simulink library "casper_library_delays"  (Simulink 7.2)
settings: Solver=ode45  SolverMode=SingleTasking  StartTime=0.0  StopTime=10.0  RelTol=1e-3
libraries: xbsIndex_r4 x388, casper_library_misc x16, casper_library_delays x16, xbsReplacements_r4 x5, casper_library_multipliers x4
(part 2 of 5)

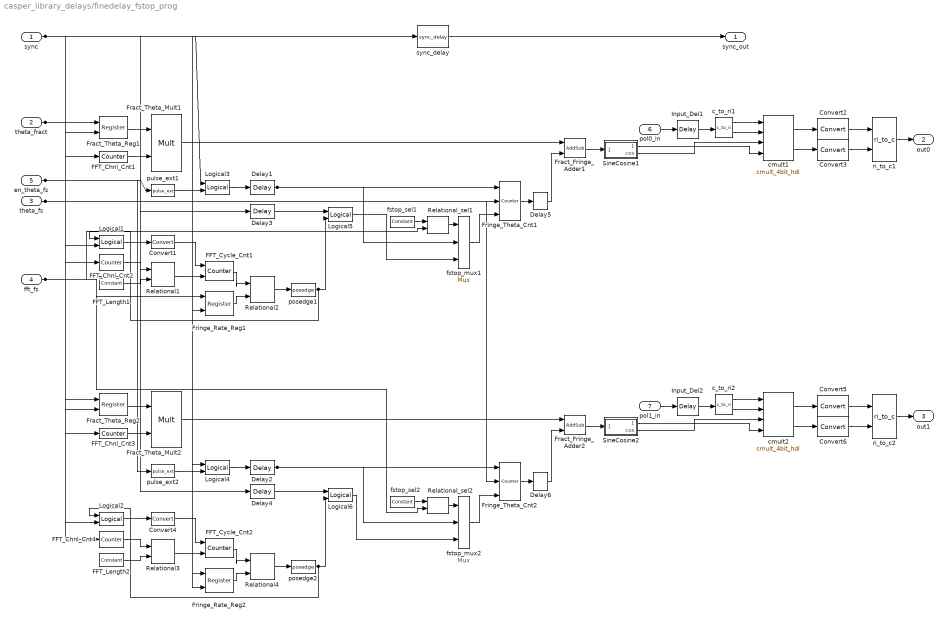
== system casper_library_delays/finedelay_fstop_prog ==
  sync : Inport
  theta_fract : Inport  Port=2
  theta_fs : Inport  Port=3
  fft_fs : Inport  Port=4
  en_theta_fs : Inport  Port=5
  pol0_in : Inport  Port=6
  pol1_in : Inport  Port=7
  Convert1 : xbsIndex_r4/Convert  gui_display_data_type=Fixed-point  arith_type=Boolean  n_bits=16  bin_pt=14  float_type=Single  exp_bits=8  fraction_bits=24  quantization=Truncate  overflow=Wrap  en=off  latency=0  dbl_ovrd=off  pipeline=off  block_type=convert
      settings: block_version=10.1.3
  Convert{2..3,5..6} (4 alike) : xbsIndex_r4/Convert  gui_display_data_type=Fixed-point  arith_type="Signed  (2's comp)"  n_bits=fft_bits  bin_pt=fft_bits-1  float_type=Single  exp_bits=8  fraction_bits=24  quantization=Truncate  overflow=Wrap  en=off  latency=0  dbl_ovrd=off  pipeline=off  block_type=convert
      settings: block_version=10.1.3
  Convert4 : xbsIndex_r4/Convert  gui_display_data_type=Fixed-point  arith_type=Boolean  n_bits=16  bin_pt=14  float_type=Single  exp_bits=8  fraction_bits=24  quantization=Truncate  overflow=Wrap  en=off  latency=0  dbl_ovrd=off  pipeline=off  block_type=convert
      settings: block_version=10.1.3
  Delay{1..4} (4 alike) : xbsIndex_r4/Delay  rst=off  infoeditControl=Selection of Reset will increase slice count due to use of real FFs and instead of SRLs  en=off  latency=1  dbl_ovrd=off  reg_retiming=off  block_type=delay
  Delay5 : xbsIndex_r4/Delay  rst=off  infoeditControl=Selection of Reset will increase slice count due to use of real FFs and instead of SRLs  en=off  latency=2  dbl_ovrd=off  reg_retiming=off  block_type=delay
  Delay6 : xbsIndex_r4/Delay  rst=off  infoeditControl=Selection of Reset will increase slice count due to use of real FFs and instead of SRLs  en=off  latency=2  dbl_ovrd=off  reg_retiming=off  block_type=delay
  FFT_Chnl_Cnt1 : xbsIndex_r4/Counter  cnt_type=Free Running  cnt_to=Inf  operation=Up  start_count=0  cnt_by_val=2  arith_type=Unsigned  n_bits=9  bin_pt=0  load_pin=off  rst=on  en=off  explicit_period=on  period=1  dbl_ovrd=off  use_behavioral_HDL=off  implementation=Fabric  use_rpm=off  block_type=counter
  FFT_Chnl_Cnt2 : xbsIndex_r4/Counter  cnt_type=Free Running  cnt_to=Inf  operation=Up  start_count=0  cnt_by_val=1  arith_type=Unsigned  n_bits=8  bin_pt=0  load_pin=off  rst=on  en=off  explicit_period=on  period=1  dbl_ovrd=off  use_behavioral_HDL=off  implementation=Fabric  use_rpm=off  block_type=counter
  FFT_Chnl_Cnt3 : xbsIndex_r4/Counter  cnt_type=Free Running  cnt_to=Inf  operation=Up  start_count=1  cnt_by_val=2  arith_type=Unsigned  n_bits=9  bin_pt=0  load_pin=off  rst=on  en=off  explicit_period=on  period=1  dbl_ovrd=off  use_behavioral_HDL=off  implementation=Fabric  use_rpm=off  block_type=counter
  FFT_Chnl_Cnt4 : xbsIndex_r4/Counter  cnt_type=Free Running  cnt_to=Inf  operation=Up  start_count=0  cnt_by_val=1  arith_type=Unsigned  n_bits=8  bin_pt=0  load_pin=off  rst=on  en=off  explicit_period=on  period=1  dbl_ovrd=off  use_behavioral_HDL=off  implementation=Fabric  use_rpm=off  block_type=counter
  FFT_Cycle_Cnt1 : xbsIndex_r4/Counter  cnt_type=Free Running  cnt_to=Inf  operation=Up  start_count=0  cnt_by_val=1  arith_type=Unsigned  n_bits=12  bin_pt=0  load_pin=off  rst=on  en=on  explicit_period=on  period=1  dbl_ovrd=off  use_behavioral_HDL=off  implementation=Fabric  use_rpm=off  block_type=counter
  FFT_Cycle_Cnt2 : xbsIndex_r4/Counter  cnt_type=Free Running  cnt_to=Inf  operation=Up  start_count=0  cnt_by_val=1  arith_type=Unsigned  n_bits=12  bin_pt=0  load_pin=off  rst=on  en=on  explicit_period=on  period=1  dbl_ovrd=off  use_behavioral_HDL=off  implementation=Fabric  use_rpm=off  block_type=counter
  FFT_Length1 : xbsIndex_r4/Constant  const=255  gui_display_data_type=Fixed-point  arith_type=Unsigned  n_bits=8  bin_pt=0  preci_type=Single  exp_width=8  frac_width=24  explicit_period=on  period=1  equ=P=C  opselect=C  inp2=PCIN>>17  opr=+  inp1=P  carry=CIN  dbl_ovrd=off  block_type=constant
  FFT_Length2 : xbsIndex_r4/Constant  const=255  gui_display_data_type=Fixed-point  arith_type=Unsigned  n_bits=8  bin_pt=0  preci_type=Single  exp_width=8  frac_width=24  explicit_period=on  period=1  equ=P=C  opselect=C  inp2=PCIN>>17  opr=+  inp1=P  carry=CIN  dbl_ovrd=off  block_type=constant
  Fract_Fringe_Adder1 : xbsIndex_r4/AddSub  mode=Addition  use_carryin=off  use_carryout=off  en=off  latency=2  precision=User Defined  arith_type=Unsigned  n_bits=14  bin_pt=0  quantization=Truncate  overflow=Wrap  dbl_ovrd=off  use_behavioral_HDL=off  hw_selection=Fabric  pipelined=off  use_rpm=on  block_type=addsub
      settings: block_version=10.1.3
  Fract_Fringe_Adder2 : xbsIndex_r4/AddSub  mode=Addition  use_carryin=off  use_carryout=off  en=off  latency=2  precision=User Defined  arith_type=Unsigned  n_bits=14  bin_pt=0  quantization=Truncate  overflow=Wrap  dbl_ovrd=off  use_behavioral_HDL=off  hw_selection=Fabric  pipelined=off  use_rpm=on  block_type=addsub
      settings: block_version=10.1.3
  Fract_Theta_Mult1 : xbsIndex_r4/Mult  precision=User Defined  arith_type=Unsigned  n_bits=14  bin_pt=0  quantization=Truncate  overflow=Wrap  en=off  latency=3  dbl_ovrd=off  use_behavioral_HDL=off  opt=Speed  use_embedded=on  optimum_pipeline=off  pipeline=on  use_rpm=on  placement_style=Triangular  block_type=mult
      settings: infoedit=Hardware notes: To use the internal pipeline stage of the dedicated multiplier you must select 'Pipeline for maximum performance'.  block_version=10.1.3
  Fract_Theta_Mult2 : xbsIndex_r4/Mult  precision=User Defined  arith_type=Unsigned  n_bits=14  bin_pt=0  quantization=Truncate  overflow=Wrap  en=off  latency=3  dbl_ovrd=off  use_behavioral_HDL=off  opt=Speed  use_embedded=on  optimum_pipeline=off  pipeline=on  use_rpm=on  placement_style=Triangular  block_type=mult
      settings: infoedit=Hardware notes: To use the internal pipeline stage of the dedicated multiplier you must select 'Pipeline for maximum performance'.  block_version=10.1.3
  Fract_Theta_Reg1 : xbsIndex_r4/Register  init=0  rst=off  en=on  dbl_ovrd=off  block_type=register
  Fract_Theta_Reg2 : xbsIndex_r4/Register  init=0  rst=off  en=on  dbl_ovrd=off  block_type=register
  Fringe_Rate_Reg1 : xbsIndex_r4/Register  init=0  rst=off  en=on  dbl_ovrd=off  block_type=register
  Fringe_Rate_Reg2 : xbsIndex_r4/Register  init=0  rst=off  en=on  dbl_ovrd=off  block_type=register
  Fringe_Theta_Cnt1 : xbsIndex_r4/Counter  cnt_type=Free Running  cnt_to=Inf  operation=Up  start_count=0  cnt_by_val=1  arith_type=Unsigned  n_bits=14  bin_pt=0  load_pin=on  rst=off  en=on  explicit_period=on  period=1  dbl_ovrd=off  use_behavioral_HDL=off  implementation=Fabric  use_rpm=off  block_type=counter
  Fringe_Theta_Cnt2 : xbsIndex_r4/Counter  cnt_type=Free Running  cnt_to=Inf  operation=Up  start_count=0  cnt_by_val=1  arith_type=Unsigned  n_bits=14  bin_pt=0  load_pin=on  rst=off  en=on  explicit_period=on  period=1  dbl_ovrd=off  use_behavioral_HDL=off  implementation=Fabric  use_rpm=off  block_type=counter
  Input_Del1 : xbsIndex_r4/Delay  rst=off  infoeditControl=Selection of Reset will increase slice count due to use of real FFs and instead of SRLs  en=off  latency=7  dbl_ovrd=off  reg_retiming=off  block_type=delay
  Input_Del2 : xbsIndex_r4/Delay  rst=off  infoeditControl=Selection of Reset will increase slice count due to use of real FFs and instead of SRLs  en=off  latency=7  dbl_ovrd=off  reg_retiming=off  block_type=delay
  Logical{1..2,5..6} (4 alike) : xbsIndex_r4/Logical  logical_function=OR  inputs=2  en=off  latency=0  precision=Full  arith_type=Unsigned  n_bits=1  bin_pt=0  align_bp=on  dbl_ovrd=off  block_type=logical
  Logical3 : xbsIndex_r4/Logical  logical_function=AND  inputs=2  en=off  latency=0  precision=Full  arith_type=Unsigned  n_bits=1  bin_pt=0  align_bp=on  dbl_ovrd=off  block_type=logical
  Logical4 : xbsIndex_r4/Logical  logical_function=AND  inputs=2  en=off  latency=0  precision=Full  arith_type=Unsigned  n_bits=1  bin_pt=0  align_bp=on  dbl_ovrd=off  block_type=logical
  Relational{1..4} (4 alike) : xbsIndex_r4/Relational  mode=a=b  en=off  latency=0  dbl_ovrd=off  block_type=relational
      settings: block_version=10.1.3
  Relational_sel1 : xbsIndex_r4/Relational  mode=a!=b  en=off  latency=0  dbl_ovrd=off  block_type=relational
      settings: block_version=10.1.3
  Relational_sel2 : xbsIndex_r4/Relational  mode=a!=b  en=off  latency=0  dbl_ovrd=off  block_type=relational
      settings: block_version=10.1.3
  SineCosine1 : Subsystem  AncestorBlock=casper_library_downconverter/sincos  mask(sincos){func=sine and cosine, neg_sin=off, neg_cos=off, symmetric=off, handle_sync=off, depth_bits=14, bit_width=18, bram_latency=2}
      mask prompts: func "Function"; neg_sin "Negative sine"; neg_cos "Negative cosine"; symmetric "Symmetric output"; handle_sync "Handle sync"; depth_bits "Lookup table depth (2^?)"; bit_width "Output bit width"; bram_latency "BRAM latency"
      mask init:
      | sincos_init(gcb, ...
      |     'func', func, ...
      |     'neg_sin', neg_sin, ...
      |     'neg_cos', neg_cos, ...
      |     'symmetric', symmetric, ...
      |     'handle_sync', handle_sync, ...
      |     'depth_bits', depth_bits, ...
      |     'bit_width', bit_width, ...
      |     'bram_latency', bram_latency);
      mask StyleString: popup(cosine|sine|sine and cosine),checkbox,checkbox,checkbox,checkbox,edit,edit,edit
  SineCosine2 : Subsystem  AncestorBlock=casper_library_downconverter/sincos  mask(sincos){func=sine and cosine, neg_sin=off, neg_cos=off, symmetric=off, handle_sync=off, depth_bits=14, bit_width=18, bram_latency=2}
      mask prompts: func "Function"; neg_sin "Negative sine"; neg_cos "Negative cosine"; symmetric "Symmetric output"; handle_sync "Handle sync"; depth_bits "Lookup table depth (2^?)"; bit_width "Output bit width"; bram_latency "BRAM latency"
      mask init: same as casper_library_delays/finedelay_fstop_prog/SineCosine1
      mask StyleString: popup(cosine|sine|sine and cosine),checkbox,checkbox,checkbox,checkbox,edit,edit,edit
  c_to_ri1 : casper_library_misc/c_to_ri  n_bits=18  bin_pt=17
  c_to_ri2 : casper_library_misc/c_to_ri  n_bits=18  bin_pt=17
  cmult1 : casper_library_multipliers/cmult_4bit_hdl  mult_latency=2  add_latency=0
  cmult2 : casper_library_multipliers/cmult_4bit_hdl  mult_latency=2  add_latency=0
  fstop_mux1 : xbsIndex_r4/Mux  inputs=2  en=off  latency=0  precision=Full  arith_type=Unsigned  n_bits=16  bin_pt=14  quantization=Truncate  overflow=Wrap  dbl_ovrd=off  block_type=mux
  fstop_mux2 : xbsIndex_r4/Mux  inputs=2  en=off  latency=0  precision=Full  arith_type=Unsigned  n_bits=16  bin_pt=14  quantization=Truncate  overflow=Wrap  dbl_ovrd=off  block_type=mux
  fstop_sel1 : xbsIndex_r4/Constant  const=0  gui_display_data_type=Fixed-point  arith_type=Unsigned  n_bits=12  bin_pt=0  preci_type=Single  exp_width=8  frac_width=24  explicit_period=on  period=1  equ=P=C  opselect=C  inp2=PCIN>>17  opr=+  inp1=P  carry=CIN  dbl_ovrd=off  block_type=constant
  fstop_sel2 : xbsIndex_r4/Constant  const=0  gui_display_data_type=Fixed-point  arith_type=Unsigned  n_bits=12  bin_pt=0  preci_type=Single  exp_width=8  frac_width=24  explicit_period=on  period=1  equ=P=C  opselect=C  inp2=PCIN>>17  opr=+  inp1=P  carry=CIN  dbl_ovrd=off  block_type=constant
  posedge1 : casper_library_misc/posedge  Tag=Rising Edge Detector
  posedge2 : casper_library_misc/posedge  Tag=Rising Edge Detector
  pulse_ext1 : casper_library_misc/pulse_ext  pulse_len=2^27
  pulse_ext2 : casper_library_misc/pulse_ext  pulse_len=2^27
  ri_to_c1 : casper_library_misc/ri_to_c
  ri_to_c2 : casper_library_misc/ri_to_c
  sync_delay : casper_library_delays/sync_delay  DelayLen=3+4+2
  sync_out : Outport
  out0 : Outport  Port=2
  out1 : Outport  Port=3
  wires:
  sync/1 -> sync_delay/1, Fract_Theta_Reg1/2, FFT_Chnl_Cnt1/1, Logical3/1, Logical1/2, FFT_Chnl_Cnt2/1, Fringe_Rate_Reg1/2, Delay3/1, Fract_Theta_Reg2/2, FFT_Chnl_Cnt3/1, Logical4/1, Logical2/2, FFT_Chnl_Cnt4/1, Fringe_Rate_Reg2/2, Delay4/1
  sync_delay/1 -> sync_out/1
  theta_fract/1 -> Fract_Theta_Reg1/1, Fract_Theta_Reg2/1
  Fract_Theta_Reg1/1 -> Fract_Theta_Mult1/1
  FFT_Chnl_Cnt1/1 -> Fract_Theta_Mult1/2
  en_theta_fs/1 -> pulse_ext1/1, pulse_ext2/1
  posedge1/1 -> Logical1/1, Logical5/2
  Logical1/1 -> Convert1/1
  FFT_Chnl_Cnt2/1 -> Relational1/1
  FFT_Length1/1 -> Relational1/2
  Convert1/1 -> FFT_Cycle_Cnt1/1
  Relational1/1 -> FFT_Cycle_Cnt1/2
  fft_fs/1 -> Fringe_Rate_Reg1/1, Relational_sel1/2, Fringe_Rate_Reg2/1, Relational_sel2/2
  FFT_Cycle_Cnt1/1 -> Relational2/1
  Fringe_Rate_Reg1/1 -> Relational2/2
  Relational2/1 -> posedge1/1
  pulse_ext1/1 -> Logical3/2
  Logical3/1 -> Delay1/1
  Delay1/1 -> Fringe_Theta_Cnt1/1, fstop_mux1/2
  theta_fs/1 -> Fringe_Theta_Cnt1/2, Fringe_Theta_Cnt2/2
  Delay3/1 -> Logical5/1
  fstop_sel1/1 -> Relational_sel1/1
  Relational_sel1/1 -> fstop_mux1/1
  Logical5/1 -> fstop_mux1/3
  fstop_mux1/1 -> Fringe_Theta_Cnt1/3
  Fract_Theta_Mult1/1 -> Fract_Fringe_Adder1/1
  Fringe_Theta_Cnt1/1 -> Delay5/1
  Delay5/1 -> Fract_Fringe_Adder1/2
  Fract_Fringe_Adder1/1 -> SineCosine1/1(theta)
  pol0_in/1 -> Input_Del1/1
  Input_Del1/1 -> c_to_ri1/1
  c_to_ri1/1 -> cmult1/1
  c_to_ri1/2 -> cmult1/2
  SineCosine1/2(cos) -> cmult1/3
  SineCosine1/1(sine) -> cmult1/4
  cmult1/1 -> Convert2/1
  cmult1/2 -> Convert3/1
  Convert2/1 -> ri_to_c1/1
  Convert3/1 -> ri_to_c1/2
  ri_to_c1/1 -> out0/1
  Fract_Theta_Reg2/1 -> Fract_Theta_Mult2/1
  FFT_Chnl_Cnt3/1 -> Fract_Theta_Mult2/2
  posedge2/1 -> Logical2/1, Logical6/2
  Logical2/1 -> Convert4/1
  FFT_Chnl_Cnt4/1 -> Relational3/1
  FFT_Length2/1 -> Relational3/2
  Convert4/1 -> FFT_Cycle_Cnt2/1
  Relational3/1 -> FFT_Cycle_Cnt2/2
  FFT_Cycle_Cnt2/1 -> Relational4/1
  Fringe_Rate_Reg2/1 -> Relational4/2
  Relational4/1 -> posedge2/1
  pulse_ext2/1 -> Logical4/2
  Logical4/1 -> Delay2/1
  Delay2/1 -> Fringe_Theta_Cnt2/1, fstop_mux2/2
  Delay4/1 -> Logical6/1
  fstop_sel2/1 -> Relational_sel2/1
  Relational_sel2/1 -> fstop_mux2/1
  Logical6/1 -> fstop_mux2/3
  fstop_mux2/1 -> Fringe_Theta_Cnt2/3
  Fract_Theta_Mult2/1 -> Fract_Fringe_Adder2/1
  Fringe_Theta_Cnt2/1 -> Delay6/1
  Delay6/1 -> Fract_Fringe_Adder2/2
  Fract_Fringe_Adder2/1 -> SineCosine2/1(theta)
  pol1_in/1 -> Input_Del2/1
  Input_Del2/1 -> c_to_ri2/1
  c_to_ri2/1 -> cmult2/1
  c_to_ri2/2 -> cmult2/2
  SineCosine2/2(cos) -> cmult2/3
  SineCosine2/1(sine) -> cmult2/4
  cmult2/1 -> Convert5/1
  cmult2/2 -> Convert6/1
  Convert5/1 -> ri_to_c2/1
  Convert6/1 -> ri_to_c2/2
  ri_to_c2/1 -> out1/1

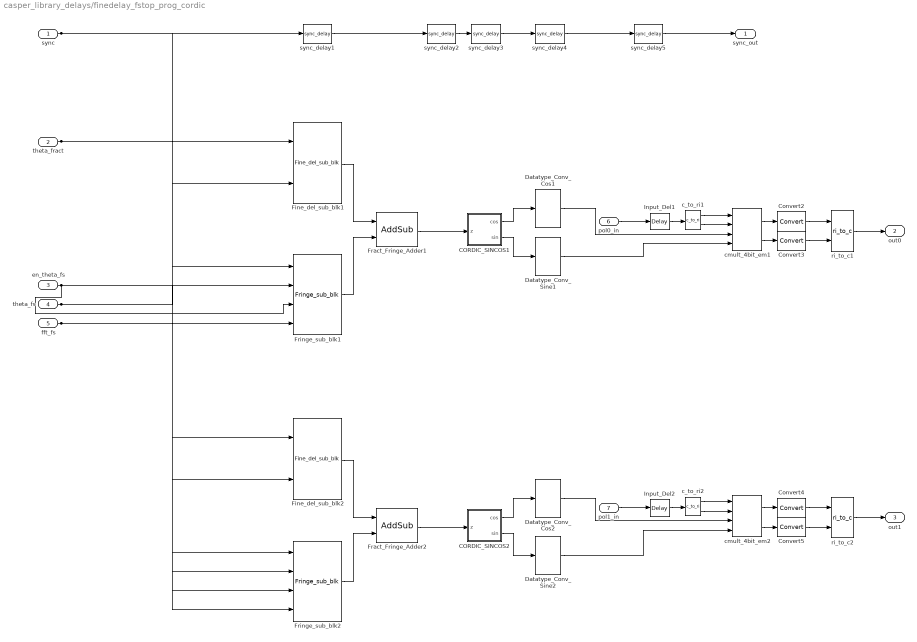
== system casper_library_delays/finedelay_fstop_prog_cordic ==
  sync : Inport
  theta_fract : Inport  Port=2
  en_theta_fs : Inport  Port=3
  theta_fs : Inport  Port=4
  fft_fs : Inport  Port=5
  pol0_in : Inport  Port=6
  pol1_in : Inport  Port=7
  CORDIC_SINCOS1 : Subsystem  mask(Xilinx CORDIC SINCOS){stages=9, pe_nbits=20, pe_binpt=17, pipeline_x=ones(1,9), prev_stages=9, pipeline=[1  1  1  1  1  1  1  1  1]}
      mask prompts: stages "Number of Processing Elements (integer value starting from 1)"; pe_nbits "Input Data Width"; pe_binpt "Input Binary Point Position"; pipeline_x "Latency for each Processing Element [1 0 0 1]"; prev_stages "Previous Number of Stages"; pipeline "Previous Pipeline Values"
      mask help: A parallel implementation, circular rotation mode CORDIC processor for calculating Sine and Cosine of input angle z. The number of iteration stages (and resultant output accuracy) and the processor arithmetic precision are controlled by the mask customization.
      mask init:
      | [bg,fg] = xlcmap('XBlock',0);
      | iPos = get_param(gcb,'Position');
      | iWidth=iPos(3)-iPos(1); iHeight=iPos(4)-iPos(2);
      | iCx=iWidth/2;
      | iCy=iHeight/2;
      | [logoX, logoY] = xlogo(iPos);
      | sav_gcb=gcb;
      | stages = round(sum(abs(stages)));
      | if (stages == 0)
      | 	stages = prev_stages;
      | end
      | x = zeros(1,stages);
      | pipe_size = max(size(pipeline_x));
      | if pipe_size >= stages
      | 	x(1,1:stages) = pipeline_x(1,1:stages);
      | else
      | 	x(1,1:pipe_size) = pipeline_x(1,1:pipe_size);
      | end
      | 
      | if (stages ~=prev_stages)
      | 	pipeline=x;
      | 	cordic_pe = find_system(gcb, 'lookUnderMasks', 'all', 'FollowLinks','on','masktype', 'CORDIC parallel PE');
      |     
      |   a=find_system(cordic_pe{1}, 'lookUnderMasks', 'all', 'FollowLinks','on','masktype', 'CORDIC iteration PE');
      |   for i= 2:length(a)
      |     for j=1:3
      | 	  delete_line(cordic_pe{1}, ['CORDIC PE' int2str(i-1) '/' int2str(j)], ['CORDIC PE' int2str(i) '/' int2str(j)]);
      |     end
      |   end
      |     if length(a)>0,
      |       delete_line(cordic_pe{1}, 'x/1', 'CORDIC PE1/1');
      |       delete_line(cordic_pe{1}, 'y/1', 'CORDIC PE1/2');
      |       delete_line(cordic_pe{1}, 'z/1', 'CORDIC PE1/3');
      |       delete_line(cordic_pe{1}, ['CORDIC PE' int2str(length(a)) '/1'],'X/1');
      |       delete_line(cordic_pe{1}, ['CORDIC PE' int2str(length(a)) '/2'],'Y/1');
      |       delete_line(cordic_pe{1}, ['CORDIC PE' int2str(length(a)) '/3'],'Terminator/1');
      |     elseif length(a)==0
      |       temp_port=get_param([cordic_pe{1} '/x'],'porthandles');
      |       temp_line=get_param(temp_port.Outport,'line');
      |       if temp_line>=0  delete_line(temp_line); end
      |       temp_port=get_param([cordic_pe{1} '/y'],'porthandles');
      |       temp_line=get_param(temp_port.Outport,'line');
      |       if temp_line>=0  delete_line(temp_line); end
      |       temp_port=get_param([cordic_pe{1} '/z'],'porthandles');
      |       temp_line=get_param(temp_port.Outport,'line');
      |       if temp_line>=0  delete_line(temp_line); end
      |     end
      | 
      |     for i=2:length(a)
      |       delete_block(a{i});
      |     end
      |     for i=2:stages,
      |         add_block([cordic_pe{1} '/CORDIC PE1'], [cordic_pe{1} '/CORDIC PE' int2str(i)], 'ii', int2str(i-1),'pe_nbits', 'pe_nbits','pe_binpt', 'pe_binpt','pipeline',['pipeline(1,' int2str(i) ')'],'position',[150+(i-1)*125, 70, 205+(i-1)*125, 130]);
      |     end
      | 
      |     for i= 2:stages,
      |       for j=1:3
      | 		add_line(cordic_pe{1}, ['CORDIC PE' int2str(i-1) '/' int2str(j)], ['CORDIC PE' int2str(i) '/' int2str(j)], 'autorouting', 'on');
      |       end
      |     end
      | 
      |     if stages==0
      |       add_line(cordic_pe{1}, 'x/1', 'X/1', 'autorouting', 'on');
      |       add_line(cordic_pe{1}, 'y/1', 'Terminator/1', 'autorouting', 'on');
      |       add_line(cordic_pe{1}, 'z/1', 'Z/1', 'autorouting', 'on');
      |     elseif stages>0
      |       add_line(cordic_pe{1}, 'x/1', 'CORDIC PE1/1', 'autorouting', 'on');
      |       add_line(cordic_pe{1}, 'y/1', 'CORDIC PE1/2', 'autorouting', 'on');
      |       add_line(cordic_pe{1}, 'z/1', 'CORDIC PE1/3', 'autorouting', 'on');
      | 
      |       set_param([cordic_pe{1} '/' 'X'], 'Position', [150+stages*125, 72, 180+stages*125, 86]);
      |       set_param([cordic_pe{1} '/' 'Y'], 'Position', [210+stages*125, 92, 225+stages*125, 108]);
      |       set_param([cordic_pe{1} '/' 'Terminator'], 'Position', [240+stages*125, 113, 270+stages*125, 127]);
      | 
      |       add_line(cordic_pe{1}, ['CORDIC PE' int2str(stages) '/1'], 'X/1', 'autorouting', 'on');
      |       add_line(cordic_pe{1}, ['CORDIC PE' int2str(stages) '/2'], 'Y/1', 'autorouting', 'on');
      |       add_line(cordic_pe{1}, ['CORDIC PE' int2str(stages) '/3'],'Terminator/1', 'autorouting', 'on');
      | 
      |       % force a "compile" of the constituent constant blocks to
      |       % workaround a data propagation problem
      |       find_system(cordic_pe{1}, 'lookUnderMasks', 'all', 'FollowLinks', 'on', 'MaskType','Xilinx Constant Block');
      |   end
      | 	set_param(sav_gcb, 'prev_stages', int2str(stages));
      | 	set_param(sav_gcb, 'pipeline', [ '[' int2str(x) ']']);
      | else
      | 	if (sum(pipeline~=x))
      | 		set_param(gcb, 'pipeline', [ '[' int2str(x) ']']);
      | 	end
      | end
      | str = sprintf('-%d',sum(x) + 3);
      settings: CopyFcn=set_param(gcb, 'MaskSelfModifiable', 'on', 'LinkStatus', 'none');
      mask Help: eval('');xlDoc('-book','sysgen','-topic','CORDIC_SINCOS');
      mask Display:
      | patch([0 iWidth iWidth 0],[0 0 iHeight iHeight] , bg);
      | patch(logoX,logoY , fg);
      | text(iCx-6,iCy,'z');
      | text(iCx,iCy+4,str);
      | port_label('input',1,'z');
      | port_label('output',1,'cos');
      | port_label('output',2,'sin');
      | plot([0 0 iWidth iWidth 0], [0 iHeight iHeight 0 0]);
  CORDIC_SINCOS2 : Subsystem  mask(Xilinx CORDIC SINCOS){stages=9, pe_nbits=20, pe_binpt=17, pipeline_x=ones(1,9), prev_stages=9, pipeline=[1  1  1  1  1  1  1  1  1]}
      mask prompts: stages "Number of Processing Elements (integer value starting from 1)"; pe_nbits "Input Data Width"; pe_binpt "Input Binary Point Position"; pipeline_x "Latency for each Processing Element [1 0 0 1]"; prev_stages "Previous Number of Stages"; pipeline "Previous Pipeline Values"
      mask help: A parallel implementation, circular rotation mode CORDIC processor for calculating Sine and Cosine of input angle z. The number of iteration stages (and resultant output accuracy) and the processor arithmetic precision are controlled by the mask customization.
      mask init: same as casper_library_delays/finedelay_fstop_prog_cordic/CORDIC_SINCOS1
      settings: CopyFcn=set_param(gcb, 'MaskSelfModifiable', 'on', 'LinkStatus', 'none');
      mask Help: eval('');xlDoc('-book','sysgen','-topic','CORDIC_SINCOS');
      mask Display:
      | patch([0 iWidth iWidth 0],[0 0 iHeight iHeight] , bg);
      | patch(logoX,logoY , fg);
      | text(iCx-6,iCy,'z');
      | text(iCx,iCy+4,str);
      | port_label('input',1,'z');
      | port_label('output',1,'cos');
      | port_label('output',2,'sin');
      | plot([0 0 iWidth iWidth 0], [0 iHeight iHeight 0 0]);
  Convert{2..5} (4 alike) : xbsIndex_r4/Convert  gui_display_data_type=Fixed-point  arith_type="Signed  (2's comp)"  n_bits=fft_bits  bin_pt=fft_bits-1  float_type=Single  exp_bits=8  fraction_bits=24  quantization=Truncate  overflow=Wrap  en=off  latency=0  dbl_ovrd=off  pipeline=off  block_type=convert
      settings: block_version=10.1.3
  Datatype_Conv_Cos1 : casper_library_delays/Datatype_Conv_Cos  theta_binary_bits=17  fft_bits=18
  Datatype_Conv_Cos2 : casper_library_delays/Datatype_Conv_Cos  theta_binary_bits=17  fft_bits=18
  Datatype_Conv_Sine1 : casper_library_delays/Datatype_Conv_Sine  theta_binary_bits=17  fft_bits=18
  Datatype_Conv_Sine2 : casper_library_delays/Datatype_Conv_Sine  theta_binary_bits=17  fft_bits=18
  Fine_del_sub_blk1 : casper_library_delays/Fine_del_sub_blk  fft_len=1024  theta_bits=20  theta_binary_bits=17
  Fine_del_sub_blk2 : casper_library_delays/Fine_del_sub_blk  fft_len=1024  theta_bits=20  theta_binary_bits=17
  Fract_Fringe_Adder1 : xbsIndex_r4/AddSub  mode=Addition  use_carryin=off  use_carryout=off  en=off  latency=2  precision=User Defined  arith_type="Signed  (2's comp)"  n_bits=20  bin_pt=17  quantization=Truncate  overflow=Wrap  dbl_ovrd=off  use_behavioral_HDL=off  hw_selection=Fabric  pipelined=off  use_rpm=on  block_type=addsub
      settings: block_version=10.1.3
  Fract_Fringe_Adder2 : xbsIndex_r4/AddSub  mode=Addition  use_carryin=off  use_carryout=off  en=off  latency=2  precision=User Defined  arith_type="Signed  (2's comp)"  n_bits=20  bin_pt=17  quantization=Truncate  overflow=Wrap  dbl_ovrd=off  use_behavioral_HDL=off  hw_selection=Fabric  pipelined=off  use_rpm=on  block_type=addsub
      settings: block_version=10.1.3
  Fringe_sub_blk1 : casper_library_delays/Fringe_sub_blk  fft_len=1024  theta_bits=20  theta_binary_bits=17  fft_cycle_bits=17  sync_period=134217728
  Fringe_sub_blk2 : casper_library_delays/Fringe_sub_blk  fft_len=1024  theta_bits=20  theta_binary_bits=17  fft_cycle_bits=17  sync_period=134217728
  Input_Del1 : xbsIndex_r4/Delay  rst=off  infoeditControl=Selection of Reset will increase slice count due to use of real FFs and instead of SRLs  en=off  latency=22  dbl_ovrd=off  reg_retiming=off  block_type=delay
  Input_Del2 : xbsIndex_r4/Delay  rst=off  infoeditControl=Selection of Reset will increase slice count due to use of real FFs and instead of SRLs  en=off  latency=22  dbl_ovrd=off  reg_retiming=off  block_type=delay
  c_to_ri1 : casper_library_misc/c_to_ri  n_bits=18  bin_pt=17
  c_to_ri2 : casper_library_misc/c_to_ri  n_bits=18  bin_pt=17
  cmult_4bit_em1 : casper_library_multipliers/cmult_4bit_em  mult_latency=2  add_latency=0
  cmult_4bit_em2 : casper_library_multipliers/cmult_4bit_em  mult_latency=2  add_latency=0
  ri_to_c1 : casper_library_misc/ri_to_c
  ri_to_c2 : casper_library_misc/ri_to_c
  sync_delay1 : casper_library_delays/sync_delay  DelayLen=7
  sync_delay2 : casper_library_delays/sync_delay  DelayLen=2
  sync_delay3 : casper_library_delays/sync_delay  DelayLen=12
  sync_delay4 : casper_library_delays/sync_delay  DelayLen=1
  sync_delay5 : casper_library_delays/sync_delay  DelayLen=2
  sync_out : Outport
  out0 : Outport  Port=2
  out1 : Outport  Port=3
  wires:
  sync/1 -> sync_delay1/1, Fine_del_sub_blk1/2, Fringe_sub_blk1/1, Fine_del_sub_blk2/2, Fringe_sub_blk2/1
  sync_delay1/1 -> sync_delay2/1
  sync_delay2/1 -> sync_delay3/1
  sync_delay3/1 -> sync_delay4/1
  sync_delay4/1 -> sync_delay5/1
  sync_delay5/1 -> sync_out/1
  theta_fract/1 -> Fine_del_sub_blk1/1, Fine_del_sub_blk2/1
  theta_fs/1 -> Fringe_sub_blk1/2, Fringe_sub_blk2/2
  en_theta_fs/1 -> Fringe_sub_blk1/3, Fringe_sub_blk2/3
  fft_fs/1 -> Fringe_sub_blk1/4, Fringe_sub_blk2/4
  Fine_del_sub_blk1/1 -> Fract_Fringe_Adder1/1
  Fringe_sub_blk1/1 -> Fract_Fringe_Adder1/2
  Fract_Fringe_Adder1/1 -> CORDIC_SINCOS1/1(z)
  CORDIC_SINCOS1/1(cos) -> Datatype_Conv_Cos1/1
  CORDIC_SINCOS1/2(sin) -> Datatype_Conv_Sine1/1
  pol0_in/1 -> Input_Del1/1
  Input_Del1/1 -> c_to_ri1/1
  c_to_ri1/1 -> cmult_4bit_em1/1
  c_to_ri1/2 -> cmult_4bit_em1/2
  Datatype_Conv_Cos1/1 -> cmult_4bit_em1/3
  Datatype_Conv_Sine1/1 -> cmult_4bit_em1/4
  cmult_4bit_em1/1 -> Convert2/1
  cmult_4bit_em1/2 -> Convert3/1
  Convert2/1 -> ri_to_c1/1
  Convert3/1 -> ri_to_c1/2
  ri_to_c1/1 -> out0/1
  Fine_del_sub_blk2/1 -> Fract_Fringe_Adder2/1
  Fringe_sub_blk2/1 -> Fract_Fringe_Adder2/2
  Fract_Fringe_Adder2/1 -> CORDIC_SINCOS2/1(z)
  CORDIC_SINCOS2/1(cos) -> Datatype_Conv_Cos2/1
  CORDIC_SINCOS2/2(sin) -> Datatype_Conv_Sine2/1
  pol1_in/1 -> Input_Del2/1
  Input_Del2/1 -> c_to_ri2/1
  c_to_ri2/1 -> cmult_4bit_em2/1
  c_to_ri2/2 -> cmult_4bit_em2/2
  Datatype_Conv_Cos2/1 -> cmult_4bit_em2/3
  Datatype_Conv_Sine2/1 -> cmult_4bit_em2/4
  cmult_4bit_em2/1 -> Convert4/1
  cmult_4bit_em2/2 -> Convert5/1
  Convert4/1 -> ri_to_c2/1
  Convert5/1 -> ri_to_c2/2
  ri_to_c2/1 -> out1/1

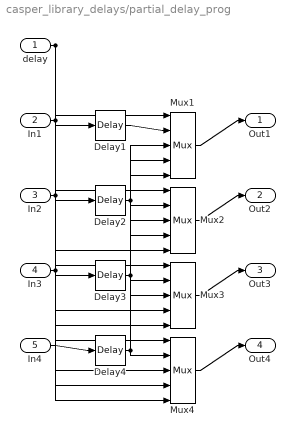
== system casper_library_delays/partial_delay_prog ==
  delay : Inport
  In1 : Inport  Port=2
  In2 : Inport  Port=3
  In3 : Inport  Port=4
  In4 : Inport  Port=5
  Delay{1..4} (4 alike) : xbsIndex_r4/Delay  rst=off  infoeditControl=Selection of Reset will increase slice count due to use of real FFs and instead of SRLs  en=off  latency=1  dbl_ovrd=off  reg_retiming=off  block_type=delay
      settings: xl_area=[0, 0, 0, 0, 0, 0, 0]  block_version=9.1.01
  Mux{1..4} (4 alike) : xbsIndex_r4/Mux  inputs=4  en=off  latency=2  precision=Full  arith_type="Signed  (2's comp)"  n_bits=8  bin_pt=2  quantization=Truncate  overflow=Wrap  dbl_ovrd=off  block_type=mux
      settings: xl_area=[0, 0, 0, 0, 0, 0, 0]  block_version=9.1.01
  Out1 : Outport
  Out2 : Outport  Port=2
  Out3 : Outport  Port=3
  Out4 : Outport  Port=4
  wires:
  In1/1 -> Delay1/1, Mux2/5, Mux3/4, Mux4/3
  Mux1/1 -> Out1/1
  delay/1 -> Mux1/1, Mux2/1, Mux3/1, Mux4/1
  Delay1/1 -> Mux1/2
  In2/1 -> Delay2/1, Mux3/5, Mux4/4
  Mux2/1 -> Out2/1
  Delay2/1 -> Mux2/2, Mux1/3
  In3/1 -> Delay3/1, Mux4/5
  Mux3/1 -> Out3/1
  Delay3/1 -> Mux3/2, Mux1/4, Mux2/3
  In4/1 -> Delay4/1
  Mux4/1 -> Out4/1
  Delay4/1 -> Mux4/2, Mux1/5, Mux2/4, Mux3/3

== system casper_library_delays/pipeline ==
  d : Inport
  Register0 : xbsIndex_r4/Register  init=0  rst=off  en=off  dbl_ovrd=off  block_type=register
      settings: block_version=11.4
  Register1 : xbsIndex_r4/Register  init=0  rst=off  en=off  dbl_ovrd=off  block_type=register
      settings: block_version=11.4
  Register2 : xbsIndex_r4/Register  init=0  rst=off  en=off  dbl_ovrd=off  block_type=register
      settings: block_version=11.4
  q : Outport
  wires:
  Register0/1 -> Register1/1
  Register1/1 -> Register2/1
  d/1 -> Register0/1
  Register2/1 -> q/1

== system casper_library_delays/sync_delay ==
  In : Inport
  Constant : xbsIndex_r4/Constant  const=1  gui_display_data_type=Fixed-point  arith_type=Unsigned  n_bits=BitWidth  bin_pt=0  preci_type=Single  exp_width=8  frac_width=24  explicit_period=on  period=1  equ=P=C  opselect=C  inp2=PCIN>>17  opr=+  inp1=P  carry=CIN  dbl_ovrd=off  block_type=constant
      settings: block_version=9.1.01
  Constant1 : xbsIndex_r4/Constant  const=0  gui_display_data_type=Fixed-point  arith_type=Unsigned  n_bits=BitWidth  bin_pt=0  preci_type=Single  exp_width=8  frac_width=24  explicit_period=on  period=1  equ=P=C  opselect=C  inp2=PCIN>>17  opr=+  inp1=P  carry=CIN  dbl_ovrd=off  block_type=constant
      settings: block_version=9.1.01
  Constant2 : xbsIndex_r4/Constant  const=DelayLen  gui_display_data_type=Fixed-point  arith_type=Unsigned  n_bits=BitWidth  bin_pt=0  preci_type=Single  exp_width=8  frac_width=24  explicit_period=on  period=1  equ=P=C  opselect=C  inp2=PCIN>>17  opr=+  inp1=P  carry=CIN  dbl_ovrd=off  block_type=constant
      settings: block_version=9.1.01
  Constant3 : xbsIndex_r4/Constant  const=UseCounter  gui_display_data_type=Fixed-point  arith_type=Unsigned  n_bits=1  bin_pt=0  preci_type=Single  exp_width=8  frac_width=24  explicit_period=on  period=1  equ=P=C  opselect=C  inp2=PCIN>>17  opr=+  inp1=P  carry=CIN  dbl_ovrd=off  block_type=constant
      settings: block_version=9.1.01
  Counter : xbsIndex_r4/Counter  cnt_type=Free Running  cnt_to=Inf  operation=Down  start_count=0  cnt_by_val=1  arith_type=Unsigned  n_bits=BitWidth  bin_pt=0  load_pin=on  rst=off  en=on  explicit_period=on  period=1  dbl_ovrd=off  use_behavioral_HDL=off  implementation=Fabric  use_rpm=on  block_type=counter
      settings: xl_area=[0, 0, 0, 0, 0, 0, 0]  block_version=9.1.01
  Logical : xbsIndex_r4/Logical  logical_function=OR  inputs=2  en=off  latency=0  precision=Full  arith_type=Unsigned  n_bits=8  bin_pt=2  align_bp=on  dbl_ovrd=off  block_type=logical
      settings: xl_area=[0, 0, 0, 0, 0, 0, 0]  block_version=9.1.01
  Mux : xbsIndex_r4/Mux  inputs=2  en=off  latency=0  precision=Full  arith_type="Signed  (2's comp)"  n_bits=8  bin_pt=2  quantization=Truncate  overflow=Wrap  dbl_ovrd=off  block_type=mux
      settings: xl_area=[0, 0, 0, 0, 0, 0, 0]  block_version=9.1.01
  Relational : xbsIndex_r4/Relational  mode=a=b  en=off  latency=0  dbl_ovrd=off  block_type=relational
      settings: xl_area=[0, 0, 0, 0, 0, 0, 0]  block_version=9.1.01
  Relational1 : xbsIndex_r4/Relational  mode=a!=b  en=off  latency=0  dbl_ovrd=off  block_type=relational
      settings: xl_area=[0, 0, 0, 0, 0, 0, 0]  block_version=9.1.01
  warn period Logical0 : xbsReplacements_r4/Warning  period=1
  warn period Relational10 : xbsReplacements_r4/Warning  period=1
  Out : Outport
  wires:
  Counter/1 -> Relational1/1, Relational/2
  Constant1/1 -> Relational1/2
  Constant/1 -> Relational/1
  Constant2/1 -> Counter/2
  In/1 -> Counter/1, Logical/1, Mux/2
  Logical/1 -> Counter/3
  Relational1/1 -> Logical/2
  Relational/1 -> Mux/3
  Constant3/1 -> Mux/1
  Mux/1 -> Out/1

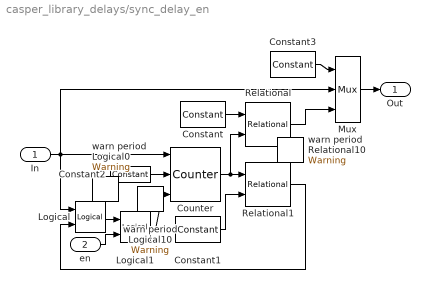
== system casper_library_delays/sync_delay_en ==
  In : Inport
  en : Inport  Port=2
  Constant : xbsIndex_r4/Constant  const=1  gui_display_data_type=Fixed-point  arith_type=Unsigned  n_bits=BitWidth  bin_pt=0  preci_type=Single  exp_width=8  frac_width=24  explicit_period=on  period=1  equ=P=C  opselect=C  inp2=PCIN>>17  opr=+  inp1=P  carry=CIN  dbl_ovrd=off  block_type=constant
      settings: block_version=9.1.01
  Constant1 : xbsIndex_r4/Constant  const=0  gui_display_data_type=Fixed-point  arith_type=Unsigned  n_bits=BitWidth  bin_pt=0  preci_type=Single  exp_width=8  frac_width=24  explicit_period=on  period=1  equ=P=C  opselect=C  inp2=PCIN>>17  opr=+  inp1=P  carry=CIN  dbl_ovrd=off  block_type=constant
      settings: block_version=9.1.01
  Constant2 : xbsIndex_r4/Constant  const=DelayLen  gui_display_data_type=Fixed-point  arith_type=Unsigned  n_bits=BitWidth  bin_pt=0  preci_type=Single  exp_width=8  frac_width=24  explicit_period=on  period=1  equ=P=C  opselect=C  inp2=PCIN>>17  opr=+  inp1=P  carry=CIN  dbl_ovrd=off  block_type=constant
      settings: block_version=9.1.01
  Constant3 : xbsIndex_r4/Constant  const=UseCounter  gui_display_data_type=Fixed-point  arith_type=Unsigned  n_bits=1  bin_pt=0  preci_type=Single  exp_width=8  frac_width=24  explicit_period=on  period=1  equ=P=C  opselect=C  inp2=PCIN>>17  opr=+  inp1=P  carry=CIN  dbl_ovrd=off  block_type=constant
      settings: block_version=9.1.01
  Counter : xbsIndex_r4/Counter  cnt_type=Free Running  cnt_to=Inf  operation=Down  start_count=0  cnt_by_val=1  arith_type=Unsigned  n_bits=BitWidth  bin_pt=0  load_pin=on  rst=off  en=on  explicit_period=on  period=1  dbl_ovrd=off  use_behavioral_HDL=off  implementation=Fabric  use_rpm=on  block_type=counter
      settings: xl_area=[0, 0, 0, 0, 0, 0, 0]  block_version=9.1.01
  Logical : xbsIndex_r4/Logical  logical_function=OR  inputs=2  en=off  latency=0  precision=Full  arith_type=Unsigned  n_bits=8  bin_pt=2  align_bp=on  dbl_ovrd=off  block_type=logical
      settings: xl_area=[0, 0, 0, 0, 0, 0, 0]  block_version=9.1.01
  Logical1 : xbsIndex_r4/Logical  logical_function=AND  inputs=2  en=off  latency=0  precision=Full  arith_type=Unsigned  n_bits=8  bin_pt=2  align_bp=on  dbl_ovrd=off  block_type=logical
      settings: xl_area=[0, 0, 0, 0, 0, 0, 0]  block_version=9.1.01
  Mux : xbsIndex_r4/Mux  inputs=2  en=off  latency=0  precision=Full  arith_type="Signed  (2's comp)"  n_bits=8  bin_pt=2  quantization=Truncate  overflow=Wrap  dbl_ovrd=off  block_type=mux
      settings: xl_area=[0, 0, 0, 0, 0, 0, 0]  block_version=9.1.01
  Relational : xbsIndex_r4/Relational  mode=a=b  en=off  latency=0  dbl_ovrd=off  block_type=relational
      settings: xl_area=[0, 0, 0, 0, 0, 0, 0]  block_version=9.1.01
  Relational1 : xbsIndex_r4/Relational  mode=a!=b  en=off  latency=0  dbl_ovrd=off  block_type=relational
      settings: xl_area=[0, 0, 0, 0, 0, 0, 0]  block_version=9.1.01
  warn period Logical0 : xbsReplacements_r4/Warning  period=1
  warn period Logical10 : xbsReplacements_r4/Warning  period=1
  warn period Relational10 : xbsReplacements_r4/Warning  period=1
  Out : Outport
  wires:
  en/1 -> Logical1/2
  Logical1/1 -> Counter/3
  Logical/1 -> Logical1/1
  Mux/1 -> Out/1
  Constant3/1 -> Mux/1
  Relational/1 -> Mux/3
  Relational1/1 -> Logical/2
  In/1 -> Mux/2, Logical/1, Counter/1
  Constant2/1 -> Counter/2
  Constant/1 -> Relational/1
  Constant1/1 -> Relational1/2
  Counter/1 -> Relational/2, Relational1/1

== system casper_library_delays/sync_delay_prog ==
  sync : Inport
  delay : Inport  Port=2
  Constant : xbsIndex_r4/Constant  const=1  gui_display_data_type=Fixed-point  arith_type=Unsigned  n_bits=MaxDelay  bin_pt=0  preci_type=Single  exp_width=8  frac_width=24  explicit_period=on  period=1  equ=P=C  opselect=C  inp2=PCIN>>17  opr=+  inp1=P  carry=CIN  dbl_ovrd=off  block_type=constant
      settings: block_version=9.1.01
  Constant1 : xbsIndex_r4/Constant  const=0  gui_display_data_type=Fixed-point  arith_type=Unsigned  n_bits=MaxDelay  bin_pt=0  preci_type=Single  exp_width=8  frac_width=24  explicit_period=on  period=1  equ=P=C  opselect=C  inp2=PCIN>>17  opr=+  inp1=P  carry=CIN  dbl_ovrd=off  block_type=constant
      settings: block_version=9.1.01
  Counter : xbsIndex_r4/Counter  cnt_type=Free Running  cnt_to=Inf  operation=Down  start_count=0  cnt_by_val=1  arith_type=Unsigned  n_bits=MaxDelay  bin_pt=0  load_pin=on  rst=off  en=on  explicit_period=on  period=1  dbl_ovrd=off  use_behavioral_HDL=off  implementation=Fabric  use_rpm=on  block_type=counter
      settings: xl_area=[0, 0, 0, 0, 0, 0, 0]  block_version=9.1.01
  Logical : xbsIndex_r4/Logical  logical_function=OR  inputs=2  en=off  latency=0  precision=Full  arith_type=Unsigned  n_bits=8  bin_pt=2  align_bp=on  dbl_ovrd=off  block_type=logical
      settings: xl_area=[0, 0, 0, 0, 0, 0, 0]  block_version=9.1.01
  Relational : xbsIndex_r4/Relational  mode=a=b  en=off  latency=0  dbl_ovrd=off  block_type=relational
      settings: xl_area=[0, 0, 0, 0, 0, 0, 0]  block_version=9.1.01
  Relational1 : xbsIndex_r4/Relational  mode=a!=b  en=off  latency=0  dbl_ovrd=off  block_type=relational
      settings: xl_area=[0, 0, 0, 0, 0, 0, 0]  block_version=9.1.01
  sync_out : Outport
  wires:
  Relational/1 -> sync_out/1
  Relational1/1 -> Logical/2
  Logical/1 -> Counter/3
  sync/1 -> Logical/1, Counter/1
  delay/1 -> Counter/2
  Constant/1 -> Relational/1
  Constant1/1 -> Relational1/2
  Counter/1 -> Relational/2, Relational1/1

== system casper_library_delays/window_delay ==
  in : Inport
  Gateway Out{2..3,55..56} (4 alike) : xbsIndex_r4/Gateway Out  inherit_from_input=off  hdl_port=on  timing_constraint=None  locs_specified=off  LOCs={}  UseAsDAC=off  DACChannel='1'  block_type=gatewayout
      settings: infoedit="Gateway out block.  Converts Xilinx fixed point inputs into ouputs of type Simulink integer, double, or fixed point.<P><P>Hardware notes:  In hardware these blocks become top level output ports or are discarded, depending on how they are configured."  xl_area=[0, 0, 0, 0, 0, 0, 0]  block_version=9.2.01
  Register : xbsIndex_r4/Register  init=0  rst=on  en=on  dbl_ovrd=off  block_type=register
      settings: xl_area=[0, 0, 0, 0, 0, 0, 0]  block_version=9.2.01
  Scope1 : Scope  NumInputPorts=4
      settings: YMin=0~0~0~-1  YMax=1~1~1~1
  negedge : Subsystem  AncestorBlock=casper_library_misc/edge_detect  mask(edge_detect){edge=Falling, polarity=Active High, x_in=[0 0.08 0.08 0.16 0.16 0.24 0.24 0.32 0.32 0.4], y_in=[1  1 -1 -1 -1 -1 -1 -1 -1 -1], x_out=[0.6 0.68 0.68 0.76 0.76 0.84 0.84 0.92 0.92 1], y_out=[-1 -1  1  1 -1 -1 -1 -1 -1 -1]}
      mask prompts: edge "Edge Type"; polarity "Output Polarity"; x_in "Input X Positions"; y_in "Input Y Positions"; x_out "Output X Positions"; y_out "Output Y Positions"
      mask help: Output is active for one-cycle after each edge of the specified type (i.e. rising, falling or both).
      mask init:
      | edge_detect_init(gcb,...
      |     'edge',edge,...
      |     'polarity',polarity,...
      |     'x_in',x_in,...
      |     'x_out',x_out,...
      |     'y_in',y_in,...
      |     'y_out',y_out);
      | 
      | x_in_num=str2num(getfield(getfield(get_param(gcb,'UserData'),'parameters'),'x_in'));
      | x_out_num=str2num(getfield(getfield(get_param(gcb,'UserData'),'parameters'),'x_out'));
      | y_in_num=str2num(getfield(getfield(get_param(gcb,'UserData'),'parameters'),'y_in'));
      | y_out_num=str2num(getfield(getfield(get_param(gcb,'UserData'),'parameters'),'y_out'));
      settings: AttributesFormatString=|
      | falling edges
      | active high
      mask Help: Output is active for one-cycle after each edge of the specified type (i.e. rising, falling, or both).  Latency is zero.
      mask StyleString: popup(Rising|Falling|Both),popup(Active High|Active Low),edit,edit,edit,edit
      mask Display:
      | plot(x_in_num,0.5+y_in_num*0.2);
      | plot(x_out_num,0.5+y_out_num*0.2);
  posedge3 : Subsystem  AncestorBlock=casper_library_misc/edge_detect  mask(edge_detect){edge=Rising, polarity=Active High, x_in=[0 0.08 0.08 0.16 0.16 0.24 0.24 0.32 0.32 0.4], y_in=[-1 -1  1  1  1  1  1  1  1  1], x_out=[0.6 0.68 0.68 0.76 0.76 0.84 0.84 0.92 0.92 1], y_out=[-1 -1  1  1 -1 -1 -1 -1 -1 -1]}
      mask prompts: edge "Edge Type"; polarity "Output Polarity"; x_in "Input X Positions"; y_in "Input Y Positions"; x_out "Output X Positions"; y_out "Output Y Positions"
      mask help: Output is active for one-cycle after each edge of the specified type (i.e. rising, falling or both).
      mask init: same as casper_library_delays/window_delay/negedge
      settings: AttributesFormatString=|
      | rising edges
      | active high
      mask Help: Output is active for one-cycle after each edge of the specified type (i.e. rising, falling, or both).  Latency is zero.
      mask StyleString: popup(Rising|Falling|Both),popup(Active High|Active Low),edit,edit,edit,edit
      mask Display:
      | plot(x_in_num,0.5+y_in_num*0.2);
      | plot(x_out_num,0.5+y_out_num*0.2);
  sync_delay : casper_library_delays/sync_delay  DelayLen=delay-1
  sync_delay1 : casper_library_delays/sync_delay  DelayLen=delay-1
  out : Outport
  wires:
  Gateway Out55/1 -> Scope1/1
  Gateway Out56/1 -> Scope1/2
  Gateway Out2/1 -> Scope1/3
  Gateway Out3/1 -> Scope1/4
  in/1 -> negedge/1(in), posedge3/1(in), Gateway Out55/1
  posedge3/1(out) -> sync_delay/1
  negedge/1(out) -> sync_delay1/1
  sync_delay/1 -> Register/1, Register/3, Gateway Out56/1
  sync_delay1/1 -> Register/2, Gateway Out2/1
  Register/1 -> out/1, Gateway Out3/1

== system casper_library_delays/delay_complex/delay1 ==
  din : Inport
  constant : xbsIndex_r4/Constant  const=1  gui_display_data_type=Fixed-point  arith_type=Boolean  n_bits=16  bin_pt=14  preci_type=Single  exp_width=8  frac_width=24  explicit_period=on  period=1  equ=P=C  opselect=C  inp2=PCIN>>17  opr=+  inp1=P  carry=CIN  dbl_ovrd=off  block_type=constant
  counter : xbsIndex_r4/Counter  cnt_type=Count Limited  cnt_to=DelayLen - bram_latency - 1  operation=Up  start_count=0  cnt_by_val=1  arith_type=Unsigned  n_bits=3  bin_pt=0  load_pin=off  rst=off  en=off  explicit_period=on  period=1  dbl_ovrd=off  use_behavioral_HDL=off  implementation=Fabric  use_rpm=off  block_type=counter
  ram : xbsIndex_r4/Single Port RAM  depth=8  initVector=0  distributed_mem=Block RAM  write_mode=Read Before Write  rst=off  init_reg=0  en=off  latency=bram_latency  dbl_ovrd=off  optimize=Area  block_type=spram
  dout : Outport
  wires:
  counter/1 -> ram/1
  din/1 -> ram/2
  constant/1 -> ram/3
  ram/1 -> dout/1

== system casper_library_delays/delay_complex/delay2 ==
  din : Inport
  constant : xbsIndex_r4/Constant  const=1  gui_display_data_type=Fixed-point  arith_type=Boolean  n_bits=16  bin_pt=14  preci_type=Single  exp_width=8  frac_width=24  explicit_period=on  period=1  equ=P=C  opselect=C  inp2=PCIN>>17  opr=+  inp1=P  carry=CIN  dbl_ovrd=off  block_type=constant
  counter : xbsIndex_r4/Counter  cnt_type=Count Limited  cnt_to=DelayLen - bram_latency - 1  operation=Up  start_count=0  cnt_by_val=1  arith_type=Unsigned  n_bits=3  bin_pt=0  load_pin=off  rst=off  en=off  explicit_period=on  period=1  dbl_ovrd=off  use_behavioral_HDL=off  implementation=Fabric  use_rpm=off  block_type=counter
  ram : xbsIndex_r4/Single Port RAM  depth=8  initVector=0  distributed_mem=Block RAM  write_mode=Read Before Write  rst=off  init_reg=0  en=off  latency=bram_latency  dbl_ovrd=off  optimize=Area  block_type=spram
  dout : Outport
  wires:
  counter/1 -> ram/1
  din/1 -> ram/2
  constant/1 -> ram/3
  ram/1 -> dout/1

== system casper_library_delays/finedelay_fstop_prog/SineCosine1 ==
  theta : Inport
  rom0 : xbsIndex_r4/ROM  depth=2^depth_bits  initVector=sin(2*pi*(0:(2^depth_bits-1))/(2^depth_bits))  distributed_mem=Block RAM  rst=off  init_reg=0  en=off  latency=bram_latency  gui_display_data_type=Fixed-point  arith_type="Signed  (2's comp)"  n_bits=bit_width  bin_pt=bit_width-1  preci_type=Single  exp_width=8  frac_width=24  dbl_ovrd=off  optimize=Area  use_rpm=on  block_type=sprom
      settings: block_version=10.1.3
  rom1 : xbsIndex_r4/ROM  depth=2^depth_bits  initVector=cos(2*pi*(0:(2^depth_bits-1))/(2^depth_bits))  distributed_mem=Block RAM  rst=off  init_reg=0  en=off  latency=bram_latency  gui_display_data_type=Fixed-point  arith_type="Signed  (2's comp)"  n_bits=bit_width  bin_pt=bit_width-1  preci_type=Single  exp_width=8  frac_width=24  dbl_ovrd=off  optimize=Area  use_rpm=on  block_type=sprom
      settings: block_version=10.1.3
  sine : Outport
  cos : Outport  Port=2
  wires:
  theta/1 -> rom0/1, rom1/1
  rom0/1 -> sine/1
  rom1/1 -> cos/1

== system casper_library_delays/finedelay_fstop_prog/SineCosine2 ==
  theta : Inport
  rom0 : xbsIndex_r4/ROM  depth=2^depth_bits  initVector=sin(2*pi*(0:(2^depth_bits-1))/(2^depth_bits))  distributed_mem=Block RAM  rst=off  init_reg=0  en=off  latency=bram_latency  gui_display_data_type=Fixed-point  arith_type="Signed  (2's comp)"  n_bits=bit_width  bin_pt=bit_width-1  preci_type=Single  exp_width=8  frac_width=24  dbl_ovrd=off  optimize=Area  use_rpm=on  block_type=sprom
      settings: block_version=10.1.3
  rom1 : xbsIndex_r4/ROM  depth=2^depth_bits  initVector=cos(2*pi*(0:(2^depth_bits-1))/(2^depth_bits))  distributed_mem=Block RAM  rst=off  init_reg=0  en=off  latency=bram_latency  gui_display_data_type=Fixed-point  arith_type="Signed  (2's comp)"  n_bits=bit_width  bin_pt=bit_width-1  preci_type=Single  exp_width=8  frac_width=24  dbl_ovrd=off  optimize=Area  use_rpm=on  block_type=sprom
      settings: block_version=10.1.3
  sine : Outport
  cos : Outport  Port=2
  wires:
  theta/1 -> rom0/1, rom1/1
  rom0/1 -> sine/1
  rom1/1 -> cos/1
